simulink model "gm_HFMA_4B_1_5_9_13"  (R2026b)
settings: Solver=FixedStepDiscrete  StopTime=stopTime  FixedStep=1.953125e-06
PreLoadFcn:
  | load('a_luts.mat')
undefined symbols (not defined in the file or in its folder): Ts
libraries: simulink x202, simulink_need_slupdate x99, hdlsllib x91
(part 15 of 20)

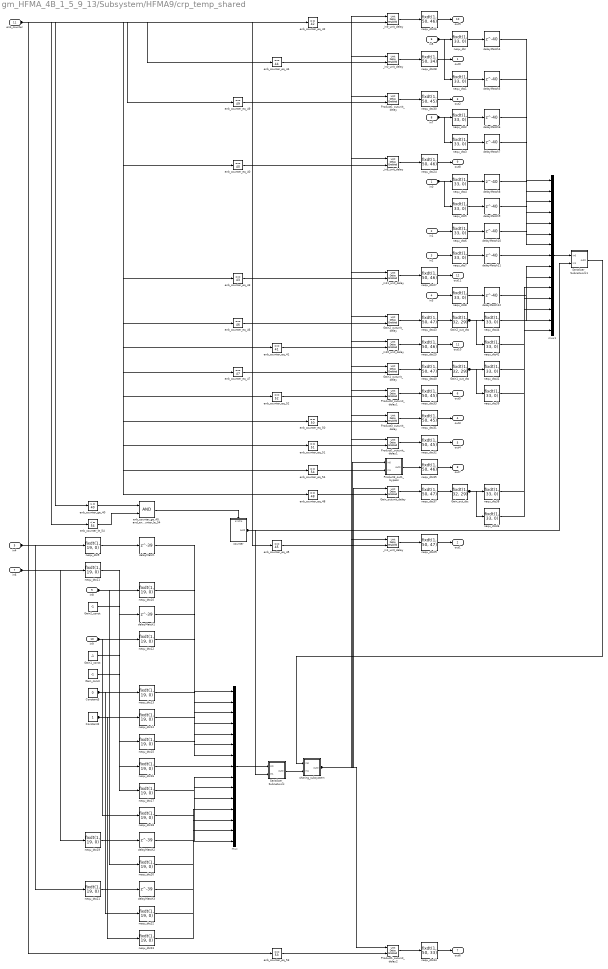
== system gm_HFMA_4B_1_5_9_13/Subsystem/HFMA9/crp_temp_shared ==
  in0 : Inport  OutDataTypeStr=fixdt(1,32,30,'DataTypeOverride', 'Off')  PortDimensions=1  SampleTime=1.953125e-06
  in1 : Inport  Port=2  OutDataTypeStr=fixdt(1,32,30,'DataTypeOverride', 'Off')  PortDimensions=1  SampleTime=1.953125e-06
  in2 : Inport  Port=3  OutDataTypeStr=fixdt(1,32,30,'DataTypeOverride', 'Off')  PortDimensions=1  SampleTime=1.953125e-06
  in3 : Inport  Port=4  OutDataTypeStr=fixdt(1,32,30,'DataTypeOverride', 'Off')  PortDimensions=1  SampleTime=1.953125e-06
  in4 : Inport  Port=5  OutDataTypeStr=fixdt(1,18,16,'DataTypeOverride', 'Off')  PortDimensions=1  SampleTime=1.953125e-06
  in5 : Inport  Port=6  OutDataTypeStr=fixdt(1,32,30,'DataTypeOverride', 'Off')  PortDimensions=1  SampleTime=1.953125e-06
  in6 : Inport  Port=7  OutDataTypeStr=fixdt(1,18,16,'DataTypeOverride', 'Off')  PortDimensions=1  SampleTime=1.953125e-06
  in7 : Inport  Port=8  OutDataTypeStr=fixdt(1,32,30,'DataTypeOverride', 'Off')  PortDimensions=1  SampleTime=1.953125e-06
  in8 : Inport  Port=9  OutDataTypeStr=fixdt(1,18,16,'DataTypeOverride', 'Off')  PortDimensions=1  SampleTime=1.953125e-06
  in9 : Inport  Port=10  OutDataTypeStr=fixdt(1,18,16,'DataTypeOverride', 'Off')  PortDimensions=1  SampleTime=1.953125e-06
  enb_counter : Inport  Port=11  OutDataTypeStr=fixdt(0,6,0,'DataTypeOverride', 'Off')  PortDimensions=1  SampleTime=1.953125e-06
  Constant2 : Constant  OutDataTypeStr=fixdt(0, 18, 17)  SampleTime=1.953125e-06
  Constant3 : Constant  Value=0  OutDataTypeStr=fixdt(1, 18, 4)  SampleTime=1.953125e-06
  Gain1_const : Constant  Value=-1  OutDataTypeStr=fixdt(1, 18, 17)  SampleTime=1.953125e-06
  Gain1_out_dtc : DataTypeConversion  OutDataTypeStr=fixdt(1, 32, 29)  SampleTime=1.953125e-06  RndMeth=Floor
  Gain1_outunit_delay : simulink_need_slupdate/Unit Delay Enabled  vinit=0.0  tsamp=-1
  Gain2_const : Constant  Value=-1  OutDataTypeStr=fixdt(1, 18, 17)  SampleTime=1.953125e-06
  Gain2_out_dtc : DataTypeConversion  OutDataTypeStr=fixdt(1, 32, 29)  SampleTime=1.953125e-06  RndMeth=Floor
  Gain2_outunit_delay : simulink_need_slupdate/Unit Delay Enabled  vinit=0.0  tsamp=-1
  Gain_const : Constant  Value=-1  OutDataTypeStr=fixdt(1, 18, 17)  SampleTime=1.953125e-06
  Gain_out_dtc : DataTypeConversion  OutDataTypeStr=fixdt(1, 32, 29)  SampleTime=1.953125e-06  RndMeth=Floor
  Gain_outunit_delay : simulink_need_slupdate/Unit Delay Enabled  vinit=0.0  tsamp=-1
  Product1_outunit_delay : simulink_need_slupdate/Unit Delay Enabled  vinit=0.0  tsamp=-1
  Product1_outunit_delay1 : simulink_need_slupdate/Unit Delay Enabled  vinit=0.0  tsamp=-1
  Product1_outunit_delay2 : simulink_need_slupdate/Unit Delay Enabled  vinit=0.0  tsamp=-1
  Product3_out1_bypass : Subsystem
  Product3_outunit_delay : simulink_need_slupdate/Unit Delay Enabled  vinit=0.0  tsamp=-1
  Product3_outunit_delay1 : simulink_need_slupdate/Unit Delay Enabled  vinit=0.0  tsamp=-1
  Serializer_Subnetwork : Subsystem
  Serializer_Subnetwork1 : Subsystem
  _in0_unit_delay : simulink_need_slupdate/Unit Delay Enabled  vinit=0.0  tsamp=-1
  _in10_unit_delay : simulink_need_slupdate/Unit Delay Enabled  vinit=0.0  tsamp=-1
  _in11_unit_delay : simulink_need_slupdate/Unit Delay Enabled  vinit=0.0  tsamp=-1
  _in1_unit_delay : simulink_need_slupdate/Unit Delay Enabled  vinit=0.0  tsamp=-1
  _in8_unit_delay : simulink_need_slupdate/Unit Delay Enabled  vinit=0.0  tsamp=-1
  _in9_unit_delay : simulink_need_slupdate/Unit Delay Enabled  vinit=0.0  tsamp=-1
  counter : Subsystem
  delayMatch{,1..3} (4 alike) : Delay  DelayLength=39  InitialCondition=0  SampleTime=1.953125e-06
  delayMatch{4..12} (9 alike) : Delay  DelayLength=40  InitialCondition=0  SampleTime=1.953125e-06
  enb_counter_eq_40 : simulink/Logic and Bit Operations/Compare To Constant  relop===  const=40  OutDataTypeStr=boolean
  enb_counter_eq_41 : simulink/Logic and Bit Operations/Compare To Constant  relop===  const=41  OutDataTypeStr=boolean
  enb_counter_eq_42 : simulink/Logic and Bit Operations/Compare To Constant  relop===  const=42  OutDataTypeStr=boolean
  enb_counter_eq_43 : simulink/Logic and Bit Operations/Compare To Constant  relop===  const=43  OutDataTypeStr=boolean
  enb_counter_eq_44 : simulink/Logic and Bit Operations/Compare To Constant  relop===  const=44  OutDataTypeStr=boolean
  enb_counter_eq_45 : simulink/Logic and Bit Operations/Compare To Constant  relop===  const=45  OutDataTypeStr=boolean
  enb_counter_eq_46 : simulink/Logic and Bit Operations/Compare To Constant  relop===  const=46  OutDataTypeStr=boolean
  enb_counter_eq_47 : simulink/Logic and Bit Operations/Compare To Constant  relop===  const=47  OutDataTypeStr=boolean
  enb_counter_eq_48 : simulink/Logic and Bit Operations/Compare To Constant  relop===  const=48  OutDataTypeStr=boolean
  enb_counter_eq_49 : simulink/Logic and Bit Operations/Compare To Constant  relop===  const=49  OutDataTypeStr=boolean
  enb_counter_eq_50 : simulink/Logic and Bit Operations/Compare To Constant  relop===  const=50  OutDataTypeStr=boolean
  enb_counter_eq_51 : simulink/Logic and Bit Operations/Compare To Constant  relop===  const=51  OutDataTypeStr=boolean
  enb_counter_eq_52 : simulink/Logic and Bit Operations/Compare To Constant  relop===  const=52  OutDataTypeStr=boolean
  enb_counter_eq_53 : simulink/Logic and Bit Operations/Compare To Constant  relop===  const=53  OutDataTypeStr=boolean
  enb_counter_eq_54 : simulink/Logic and Bit Operations/Compare To Constant  relop===  const=54  OutDataTypeStr=boolean
  enb_counter_ge_40 : simulink/Logic and Bit Operations/Compare To Constant  relop=>=  const=40  OutDataTypeStr=boolean
  enb_counter_ge_40_and_enb_counter_le_54 : Logic  AllPortsSameDT=off  OutDataTypeStr=boolean  SampleTime=1.953125e-06
  enb_counter_le_54 : simulink/Logic and Bit Operations/Compare To Constant  relop=<=  const=54  OutDataTypeStr=boolean
  mux : Mux  Inputs=15
  mux1 : Mux  Inputs=15
  nequ_dtc{,1..8,36,38..39,41..42,44} (15 alike) : DataTypeConversion  OutDataTypeStr=fixdt(1, 33, 0)  ConvertRealWorld=Stored Integer (SI)  SampleTime=1.953125e-06  SaturateOnIntegerOverflow=off  RndMeth=Floor
  nequ_dtc{9..23} (15 alike) : DataTypeConversion  OutDataTypeStr=fixdt(1, 19, 0)  ConvertRealWorld=Stored Integer (SI)  SampleTime=1.953125e-06  SaturateOnIntegerOverflow=off  RndMeth=Floor
  nequ_dtc{24..27,35} (5 alike) : DataTypeConversion  OutDataTypeStr=fixdt(1, 50, 46)  ConvertRealWorld=Stored Integer (SI)  SampleTime=1.953125e-06  SaturateOnIntegerOverflow=off  RndMeth=Floor
  nequ_dtc28 : DataTypeConversion  OutDataTypeStr=fixdt(1, 50, 34)  ConvertRealWorld=Stored Integer (SI)  SampleTime=1.953125e-06  SaturateOnIntegerOverflow=off  RndMeth=Floor
  nequ_dtc{29,37,40,43} (4 alike) : DataTypeConversion  OutDataTypeStr=fixdt(1, 50, 47)  ConvertRealWorld=Stored Integer (SI)  SampleTime=1.953125e-06  SaturateOnIntegerOverflow=off  RndMeth=Floor
  nequ_dtc{30..33} (4 alike) : DataTypeConversion  OutDataTypeStr=fixdt(1, 50, 45)  ConvertRealWorld=Stored Integer (SI)  SampleTime=1.953125e-06  SaturateOnIntegerOverflow=off  RndMeth=Floor
  nequ_dtc34 : DataTypeConversion  OutDataTypeStr=fixdt(1, 50, 33)  ConvertRealWorld=Stored Integer (SI)  SampleTime=1.953125e-06  SaturateOnIntegerOverflow=off  RndMeth=Floor
  sharing_subsystem : Subsystem
  out0 : Outport  OutDataTypeStr=fixdt(1,50,34,'DataTypeOverride', 'Off')  PortDimensions=1  SampleTime=1.953125e-06
  out1 : Outport  Port=2  OutDataTypeStr=fixdt(1,50,47,'DataTypeOverride', 'Off')  PortDimensions=1  SampleTime=1.953125e-06
  out2 : Outport  Port=3  OutDataTypeStr=fixdt(1,50,45,'DataTypeOverride', 'Off')  PortDimensions=1  SampleTime=1.953125e-06
  out3 : Outport  Port=4  OutDataTypeStr=fixdt(1,50,45,'DataTypeOverride', 'Off')  PortDimensions=1  SampleTime=1.953125e-06
  out4 : Outport  Port=5  OutDataTypeStr=fixdt(1,50,45,'DataTypeOverride', 'Off')  PortDimensions=1  SampleTime=1.953125e-06
  out5 : Outport  Port=6  OutDataTypeStr=fixdt(1,50,45,'DataTypeOverride', 'Off')  PortDimensions=1  SampleTime=1.953125e-06
  out6 : Outport  Port=7  OutDataTypeStr=fixdt(1,50,33,'DataTypeOverride', 'Off')  PortDimensions=1  SampleTime=1.953125e-06
  out7 : Outport  Port=8  OutDataTypeStr=fixdt(1,50,46,'DataTypeOverride', 'Off')  PortDimensions=1  SampleTime=1.953125e-06
  out8 : Outport  Port=9  OutDataTypeStr=fixdt(1,50,46,'DataTypeOverride', 'Off')  PortDimensions=1  SampleTime=1.953125e-06
  out9 : Outport  Port=10  OutDataTypeStr=fixdt(1,50,46,'DataTypeOverride', 'Off')  PortDimensions=1  SampleTime=1.953125e-06
  out10 : Outport  Port=11  OutDataTypeStr=fixdt(1,50,46,'DataTypeOverride', 'Off')  PortDimensions=1  SampleTime=1.953125e-06
  out11 : Outport  Port=12  OutDataTypeStr=fixdt(1,50,46,'DataTypeOverride', 'Off')  PortDimensions=1  SampleTime=1.953125e-06
  wires:
  nequ_dtc30/1 -> out2/1
  Product3_outunit_delay1/1 -> nequ_dtc33/1
  enb_counter_eq_48/1 -> Gain_outunit_delay/2
  nequ_dtc9/1 -> delayMatch/1
  Product3_out1_bypass/1(out0) -> nequ_dtc35/1
  Gain_outunit_delay/1 -> nequ_dtc37/1
  nequ_dtc11/1 -> delayMatch1/1
  Gain2_outunit_delay/1 -> nequ_dtc43/1
  nequ_dtc13/1 -> mux/5
  enb_counter_le_54/1 -> enb_counter_ge_40_and_enb_counter_le_54/2
  enb_counter_eq_50/1 -> Product3_outunit_delay/2
  nequ_dtc19/1 -> delayMatch2/1
  nequ_dtc21/1 -> delayMatch3/1
  enb_counter_ge_40/1 -> enb_counter_ge_40_and_enb_counter_le_54/1
  in3/1 -> nequ_dtc8/1
  nequ_dtc38/1 -> mux1/14
  nequ_dtc43/1 -> Gain2_out_dtc/1
  enb_counter_eq_42/1 -> _in9_unit_delay/2
  Serializer_Subnetwork/1(out0) -> sharing_subsystem/2(in1)
  delayMatch5/1 -> mux1/2
  enb_counter_eq_54/1 -> Product3_out1_bypass/2(in1)
  Gain_out_dtc/1 -> nequ_dtc36/1, nequ_dtc38/1
  in1/1 -> nequ_dtc6/1
  enb_counter_eq_51/1 -> Product1_outunit_delay1/2
  nequ_dtc44/1 -> mux1/10
  enb_counter_eq_46/1 -> Gain2_outunit_delay/2
  nequ_dtc4/1 -> delayMatch8/1
  in6/1 -> nequ_dtc11/1, nequ_dtc19/1
  nequ_dtc39/1 -> mux1/13
  nequ_dtc40/1 -> Gain1_out_dtc/1
  nequ_dtc27/1 -> out11/1
  nequ_dtc29/1 -> out1/1
  enb_counter/1 -> enb_counter_eq_53/1, enb_counter_eq_52/1, enb_counter_eq_50/1, enb_counter_eq_49/1, enb_counter_eq_48/1, enb_counter_eq_47/1, enb_counter_eq_46/1, enb_counter_eq_45/1, enb_counter_eq_41/1, enb_counter_eq_54/1, enb_counter_eq_44/1, enb_counter_eq_42/1, enb_counter_eq_40/1, enb_counter_eq_51/1, enb_counter_le_54/1, enb_counter_ge_40/1, enb_counter_eq_43/1
  nequ_dtc42/1 -> mux1/11
  nequ_dtc41/1 -> mux1/12
  delayMatch7/1 -> mux1/4
  delayMatch9/1 -> mux1/6
  Product1_outunit_delay2/1 -> nequ_dtc34/1
  Gain1_outunit_delay/1 -> nequ_dtc40/1
  nequ_dtc37/1 -> Gain_out_dtc/1
  Product3_outunit_delay/1 -> nequ_dtc31/1
  Product1_outunit_delay/1 -> nequ_dtc30/1
  nequ_dtc6/1 -> delayMatch10/1
  nequ_dtc8/1 -> delayMatch12/1
  mux1/1 -> Serializer_Subnetwork1/1(in0)
  nequ_dtc36/1 -> mux1/15
  nequ_dtc3/1 -> delayMatch7/1
  nequ_dtc5/1 -> delayMatch9/1
  delayMatch4/1 -> mux1/1
  delayMatch6/1 -> mux1/3
  delayMatch12/1 -> mux1/9
  delayMatch11/1 -> mux1/8
  Serializer_Subnetwork1/1(out0) -> sharing_subsystem/1(in0)
  delayMatch10/1 -> mux1/7
  _in1_unit_delay/1 -> nequ_dtc29/1
  delayMatch8/1 -> mux1/5
  Gain1_out_dtc/1 -> nequ_dtc41/1, nequ_dtc39/1
  nequ_dtc7/1 -> delayMatch11/1
  Gain1_const/1 -> nequ_dtc16/1
  nequ_dtc/1 -> delayMatch4/1
  sharing_subsystem/1(out0) -> Gain2_outunit_delay/1, Gain1_outunit_delay/1, Gain_outunit_delay/1, _in1_unit_delay/1, _in0_unit_delay/1, _in11_unit_delay/1, _in9_unit_delay/1, _in10_unit_delay/1, _in8_unit_delay/1, Product1_outunit_delay2/1, Product3_outunit_delay1/1, Product1_outunit_delay1/1, Product1_outunit_delay/1, Product3_out1_bypass/1(in0), Product3_outunit_delay/1
  nequ_dtc2/1 -> delayMatch6/1
  _in0_unit_delay/1 -> nequ_dtc28/1
  nequ_dtc1/1 -> delayMatch5/1
  nequ_dtc23/1 -> mux/15
  Product1_outunit_delay1/1 -> nequ_dtc32/1
  nequ_dtc28/1 -> out0/1
  _in11_unit_delay/1 -> nequ_dtc27/1
  nequ_dtc34/1 -> out6/1
  _in9_unit_delay/1 -> nequ_dtc26/1
  nequ_dtc26/1 -> out9/1
  _in10_unit_delay/1 -> nequ_dtc25/1
  nequ_dtc20/1 -> mux/12
  nequ_dtc25/1 -> out10/1
  mux/1 -> Serializer_Subnetwork/1(in0)
  _in8_unit_delay/1 -> nequ_dtc24/1
  nequ_dtc24/1 -> out8/1
  in5/1 -> nequ_dtc1/1, nequ_dtc/1
  nequ_dtc22/1 -> mux/14
  delayMatch3/1 -> mux/13
  delayMatch2/1 -> mux/11
  nequ_dtc18/1 -> mux/10
  nequ_dtc17/1 -> mux/9
  nequ_dtc16/1 -> mux/8
  nequ_dtc15/1 -> mux/7
  nequ_dtc14/1 -> mux/6
  nequ_dtc12/1 -> mux/4
  delayMatch1/1 -> mux/3
  nequ_dtc10/1 -> mux/2
  delayMatch/1 -> mux/1
  in2/1 -> nequ_dtc7/1
  nequ_dtc35/1 -> out7/1
  nequ_dtc33/1 -> out5/1
  nequ_dtc32/1 -> out4/1
  nequ_dtc31/1 -> out3/1
  Gain_const/1 -> nequ_dtc17/1
  Gain2_const/1 -> nequ_dtc15/1
  enb_counter_ge_40_and_enb_counter_le_54/1 -> counter/Enable
  Constant2/1 -> nequ_dtc14/1, nequ_dtc23/1
  counter/1(out0) -> Serializer_Subnetwork1/2(in1), Serializer_Subnetwork/2(in1)
  in9/1 -> nequ_dtc18/1, nequ_dtc12/1
  Gain2_out_dtc/1 -> nequ_dtc42/1, nequ_dtc44/1
  Constant3/1 -> nequ_dtc13/1, nequ_dtc22/1
  in0/1 -> nequ_dtc5/1, nequ_dtc4/1
  in8/1 -> nequ_dtc20/1, nequ_dtc10/1
  in7/1 -> nequ_dtc3/1, nequ_dtc2/1
  in4/1 -> nequ_dtc21/1, nequ_dtc9/1
  enb_counter_eq_53/1 -> Product1_outunit_delay2/2
  enb_counter_eq_49/1 -> Product1_outunit_delay/2
  enb_counter_eq_40/1 -> _in8_unit_delay/2
  enb_counter_eq_43/1 -> _in11_unit_delay/2
  enb_counter_eq_47/1 -> Gain1_outunit_delay/2
  enb_counter_eq_41/1 -> _in10_unit_delay/2
  enb_counter_eq_52/1 -> Product3_outunit_delay1/2
  enb_counter_eq_44/1 -> _in0_unit_delay/2
  enb_counter_eq_45/1 -> _in1_unit_delay/2

== system gm_HFMA_4B_1_5_9_13/Subsystem/HFMA9/crp_temp_shared1 ==
  in0 : Inport  OutDataTypeStr=fixdt(1,20,17,'DataTypeOverride', 'Off')  PortDimensions=1  SampleTime=1.953125e-06
  in1 : Inport  Port=2  OutDataTypeStr=fixdt(1,18,16,'DataTypeOverride', 'Off')  PortDimensions=1  SampleTime=1.953125e-06
  in2 : Inport  Port=3  OutDataTypeStr=fixdt(1,18,16,'DataTypeOverride', 'Off')  PortDimensions=1  SampleTime=1.953125e-06
  in3 : Inport  Port=4  OutDataTypeStr=fixdt(1,20,17,'DataTypeOverride', 'Off')  PortDimensions=1  SampleTime=1.953125e-06
  in4 : Inport  Port=5  OutDataTypeStr=fixdt(1,18,16,'DataTypeOverride', 'Off')  PortDimensions=1  SampleTime=1.953125e-06
  in5 : Inport  Port=6  OutDataTypeStr=fixdt(1,20,17,'DataTypeOverride', 'Off')  PortDimensions=1  SampleTime=1.953125e-06
  in6 : Inport  Port=7  OutDataTypeStr=fixdt(1,18,16,'DataTypeOverride', 'Off')  PortDimensions=1  SampleTime=1.953125e-06
  in7 : Inport  Port=8  OutDataTypeStr=fixdt(1,18,16,'DataTypeOverride', 'Off')  PortDimensions=1  SampleTime=1.953125e-06
  in8 : Inport  Port=9  OutDataTypeStr=fixdt(1,20,17,'DataTypeOverride', 'Off')  PortDimensions=1  SampleTime=1.953125e-06
  in9 : Inport  Port=10  OutDataTypeStr=fixdt(1,18,16,'DataTypeOverride', 'Off')  PortDimensions=1  SampleTime=1.953125e-06
  in10 : Inport  Port=11  OutDataTypeStr=fixdt(1,18,16,'DataTypeOverride', 'Off')  PortDimensions=1  SampleTime=1.953125e-06
  in11 : Inport  Port=12  OutDataTypeStr=fixdt(1,18,16,'DataTypeOverride', 'Off')  PortDimensions=1  SampleTime=1.953125e-06
  enb_counter : Inport  Port=13  OutDataTypeStr=fixdt(0,6,0,'DataTypeOverride', 'Off')  PortDimensions=1  SampleTime=1.953125e-06
  Product1 : Product  Inputs=**  OutDataTypeStr=fixdt(1, 38, 33)  SampleTime=1.953125e-06
  Serializer_Subnetwork : Subsystem
  Serializer_Subnetwork1 : Subsystem
  counter : Subsystem
  counter_matching_delay : Delay  DelayLength=15  InitialCondition=0  SampleTime=1.953125e-06
  delayMatch : Delay  DelayLength=15  InitialCondition=0  SampleTime=1.953125e-06
  demux : Demux  Outputs=8
  enb_counter_eq_23 : simulink/Logic and Bit Operations/Compare To Constant  relop===  const=23  OutDataTypeStr=boolean
  enb_counter_ge_1 : simulink/Logic and Bit Operations/Compare To Constant  relop=>=  const=1  OutDataTypeStr=boolean
  enb_counter_ge_16 : simulink/Logic and Bit Operations/Compare To Constant  relop=>=  const=16  OutDataTypeStr=boolean
  enb_counter_ge_16_and_enb_counter_le_23 : Logic  AllPortsSameDT=off  OutDataTypeStr=boolean  SampleTime=1.953125e-06
  enb_counter_ge_1_and_enb_counter_le_8 : Logic  AllPortsSameDT=off  OutDataTypeStr=boolean  SampleTime=1.953125e-06
  enb_counter_le_23 : simulink/Logic and Bit Operations/Compare To Constant  relop=<=  const=23  OutDataTypeStr=boolean
  enb_counter_le_8 : simulink/Logic and Bit Operations/Compare To Constant  relop=<=  const=8  OutDataTypeStr=boolean
  mux : Mux  Inputs=8
  mux1 : Mux  Inputs=8
  tapped_delay : hdlsllib/Discrete/Tapped Delay Enabled Synchronous  vinit=0  samptime=-1  NumDelays=7  DelayOrder=Oldest  includeCurrent=on
  tapped_delay_outunit_delay : simulink_need_slupdate/Unit Delay Enabled  vinit=0.0  tsamp=-1
  out0 : Outport  OutDataTypeStr=fixdt(1,38,33,'DataTypeOverride', 'Off')  PortDimensions=1  SampleTime=1.953125e-06
  out1 : Outport  Port=2  OutDataTypeStr=fixdt(1,38,33,'DataTypeOverride', 'Off')  PortDimensions=1  SampleTime=1.953125e-06
  out2 : Outport  Port=3  OutDataTypeStr=fixdt(1,38,33,'DataTypeOverride', 'Off')  PortDimensions=1  SampleTime=1.953125e-06
  out3 : Outport  Port=4  OutDataTypeStr=fixdt(1,38,33,'DataTypeOverride', 'Off')  PortDimensions=1  SampleTime=1.953125e-06
  out4 : Outport  Port=5  OutDataTypeStr=fixdt(1,38,33,'DataTypeOverride', 'Off')  PortDimensions=1  SampleTime=1.953125e-06
  out5 : Outport  Port=6  OutDataTypeStr=fixdt(1,38,33,'DataTypeOverride', 'Off')  PortDimensions=1  SampleTime=1.953125e-06
  out6 : Outport  Port=7  OutDataTypeStr=fixdt(1,38,33,'DataTypeOverride', 'Off')  PortDimensions=1  SampleTime=1.953125e-06
  out7 : Outport  Port=8  OutDataTypeStr=fixdt(1,38,33,'DataTypeOverride', 'Off')  PortDimensions=1  SampleTime=1.953125e-06
  wires:
  in10/1 -> mux1/7
  enb_counter/1 -> enb_counter_le_23/1, enb_counter_eq_23/1, enb_counter_le_8/1, enb_counter_ge_1/1, enb_counter_ge_16/1
  in5/1 -> mux/8, mux/4
  in7/1 -> mux1/5
  enb_counter_ge_1/1 -> enb_counter_ge_1_and_enb_counter_le_8/1
  enb_counter_ge_1_and_enb_counter_le_8/1 -> counter/Enable
  enb_counter_le_8/1 -> enb_counter_ge_1_and_enb_counter_le_8/2
  enb_counter_ge_16/1 -> enb_counter_ge_16_and_enb_counter_le_23/1
  enb_counter_le_23/1 -> enb_counter_ge_16_and_enb_counter_le_23/2
  in2/1 -> mux1/2
  in1/1 -> mux1/1
  in4/1 -> mux1/3
  in6/1 -> mux1/4
  in9/1 -> mux1/6
  in11/1 -> mux1/8
  enb_counter_ge_16_and_enb_counter_le_23/1 -> tapped_delay/2
  in0/1 -> mux/2, mux/1
  in3/1 -> mux/3, mux/5
  in8/1 -> mux/7, mux/6
  counter/1(out0) -> Serializer_Subnetwork1/2(in1), counter_matching_delay/1
  mux1/1 -> Serializer_Subnetwork1/1(in0)
  mux/1 -> Serializer_Subnetwork/1(in0)
  counter_matching_delay/1 -> Serializer_Subnetwork/2(in1)
  Serializer_Subnetwork1/1(out0) -> delayMatch/1
  Serializer_Subnetwork/1(out0) -> Product1/1
  demux/7 -> out6/1
  delayMatch/1 -> Product1/2
  Product1/1 -> tapped_delay/1
  enb_counter_eq_23/1 -> tapped_delay_outunit_delay/2
  tapped_delay/1 -> tapped_delay_outunit_delay/1
  tapped_delay_outunit_delay/1 -> demux/1
  demux/3 -> out2/1
  demux/1 -> out0/1
  demux/2 -> out1/1
  demux/6 -> out5/1
  demux/4 -> out3/1
  demux/5 -> out4/1
  demux/8 -> out7/1

== system gm_HFMA_4B_1_5_9_13/Subsystem/HFMA9/crp_temp_shared2 ==
  in0 : Inport  OutDataTypeStr=fixdt(1,18,15,'DataTypeOverride', 'Off')  PortDimensions=1  SampleTime=1.953125e-06
  in1 : Inport  Port=2  OutDataTypeStr=fixdt(1,18,15,'DataTypeOverride', 'Off')  PortDimensions=1  SampleTime=1.953125e-06
  in2 : Inport  Port=3  OutDataTypeStr=fixdt(1,18,15,'DataTypeOverride', 'Off')  PortDimensions=1  SampleTime=1.953125e-06
  in3 : Inport  Port=4  OutDataTypeStr=fixdt(1,18,15,'DataTypeOverride', 'Off')  PortDimensions=1  SampleTime=1.953125e-06
  in4 : Inport  Port=5  OutDataTypeStr=fixdt(1,18,16,'DataTypeOverride', 'Off')  PortDimensions=1  SampleTime=1.953125e-06
  in5 : Inport  Port=6  OutDataTypeStr=fixdt(1,18,16,'DataTypeOverride', 'Off')  PortDimensions=1  SampleTime=1.953125e-06
  in6 : Inport  Port=7  OutDataTypeStr=fixdt(1,18,14,'DataTypeOverride', 'Off')  PortDimensions=1  SampleTime=1.953125e-06
  in7 : Inport  Port=8  OutDataTypeStr=fixdt(1,18,14,'DataTypeOverride', 'Off')  PortDimensions=1  SampleTime=1.953125e-06
  in8 : Inport  Port=9  OutDataTypeStr=fixdt(1,18,14,'DataTypeOverride', 'Off')  PortDimensions=1  SampleTime=1.953125e-06
  in9 : Inport  Port=10  OutDataTypeStr=fixdt(1,18,14,'DataTypeOverride', 'Off')  PortDimensions=1  SampleTime=1.953125e-06
  enb_counter : Inport  Port=11  OutDataTypeStr=fixdt(0,6,0,'DataTypeOverride', 'Off')  PortDimensions=1  SampleTime=1.953125e-06
  Gain : Product  Inputs=**  OutDataTypeStr=fixdt(1, 36, 0)  SampleTime=1.953125e-06
  Gain1_const : Constant  Value=-1  OutDataTypeStr=fixdt(1, 18, 17)  SampleTime=1.953125e-06
  Gain_const{,1..3} (4 alike) : Constant  Value=-2  OutDataTypeStr=fixdt(1, 18, 16)  SampleTime=1.953125e-06
  Gain_const4 : Constant  Value=-1  OutDataTypeStr=fixdt(1, 18, 17)  SampleTime=1.953125e-06
  Serializer_Subnetwork : Subsystem
  Serializer_Subnetwork1 : Subsystem
  b0_1_const : Constant  Value=0.001172125339508056640625  OutDataTypeStr=fixdt(1, 18, 26)  SampleTime=1.953125e-06
  b0_1_const1 : Constant  Value=0.001172125339508056640625  OutDataTypeStr=fixdt(1, 18, 26)  SampleTime=1.953125e-06
  b0_1_const2 : Constant  Value=0.001172125339508056640625  OutDataTypeStr=fixdt(1, 18, 26)  SampleTime=1.953125e-06
  b1_1_const : Constant  Value=0.00234425067901611328125  OutDataTypeStr=fixdt(1, 18, 25)  SampleTime=1.953125e-06
  b1_1_const1 : Constant  Value=0.00234425067901611328125  OutDataTypeStr=fixdt(1, 18, 25)  SampleTime=1.953125e-06
  b1_1_const2 : Constant  Value=0.00234425067901611328125  OutDataTypeStr=fixdt(1, 18, 25)  SampleTime=1.953125e-06
  b2_1_const{,1..3} (4 alike) : Constant  Value=0.001172125339508056640625  OutDataTypeStr=fixdt(1, 18, 26)  SampleTime=1.953125e-06
  counter : Subsystem
  counter_matching_delay : Delay  DelayLength=24  InitialCondition=0  SampleTime=1.953125e-06
  delayMatch : Delay  DelayLength=23  InitialCondition=0  SampleTime=1.953125e-06
  delayMatch1 : Delay  DelayLength=23  InitialCondition=0  SampleTime=1.953125e-06
  delayMatch2 : Delay  DelayLength=24  InitialCondition=0  SampleTime=1.953125e-06
  demux : Demux  Outputs=16
  enb_counter_eq_39 : simulink/Logic and Bit Operations/Compare To Constant  relop===  const=39  OutDataTypeStr=boolean
  enb_counter_ge_24 : simulink/Logic and Bit Operations/Compare To Constant  relop=>=  const=24  OutDataTypeStr=boolean
  enb_counter_ge_24_and_enb_counter_le_39 : Logic  AllPortsSameDT=off  OutDataTypeStr=boolean  SampleTime=1.953125e-06
  enb_counter_le_15 : simulink/Logic and Bit Operations/Compare To Constant  relop=<=  const=15  OutDataTypeStr=boolean
  enb_counter_le_39 : simulink/Logic and Bit Operations/Compare To Constant  relop=<=  const=39  OutDataTypeStr=boolean
  mux : Mux  Inputs=16
  mux1 : Mux  Inputs=16
  nequ_dtc{,1..31} (32 alike) : DataTypeConversion  OutDataTypeStr=fixdt(1, 18, 0)  ConvertRealWorld=Stored Integer (SI)  SampleTime=1.953125e-06  SaturateOnIntegerOverflow=off  RndMeth=Floor
  nequ_dtc{32..35} (4 alike) : DataTypeConversion  OutDataTypeStr=fixdt(1, 36, 31)  ConvertRealWorld=Stored Integer (SI)  SampleTime=1.953125e-06  SaturateOnIntegerOverflow=off  RndMeth=Floor
  nequ_dtc36 : DataTypeConversion  OutDataTypeStr=fixdt(1, 36, 33)  ConvertRealWorld=Stored Integer (SI)  SampleTime=1.953125e-06  SaturateOnIntegerOverflow=off  RndMeth=Floor
  nequ_dtc37 : DataTypeConversion  OutDataTypeStr=fixdt(1, 36, 33)  ConvertRealWorld=Stored Integer (SI)  SampleTime=1.953125e-06  SaturateOnIntegerOverflow=off  RndMeth=Floor
  nequ_dtc{38..39,41..42,44..45,47} (7 alike) : DataTypeConversion  OutDataTypeStr=fixdt(1, 36, 40)  ConvertRealWorld=Stored Integer (SI)  SampleTime=1.953125e-06  SaturateOnIntegerOverflow=off  RndMeth=Floor
  nequ_dtc40 : DataTypeConversion  OutDataTypeStr=fixdt(1, 36, 39)  ConvertRealWorld=Stored Integer (SI)  SampleTime=1.953125e-06  SaturateOnIntegerOverflow=off  RndMeth=Floor
  nequ_dtc43 : DataTypeConversion  OutDataTypeStr=fixdt(1, 36, 39)  ConvertRealWorld=Stored Integer (SI)  SampleTime=1.953125e-06  SaturateOnIntegerOverflow=off  RndMeth=Floor
  nequ_dtc46 : DataTypeConversion  OutDataTypeStr=fixdt(1, 36, 39)  ConvertRealWorld=Stored Integer (SI)  SampleTime=1.953125e-06  SaturateOnIntegerOverflow=off  RndMeth=Floor
  tapped_delay : hdlsllib/Discrete/Tapped Delay Enabled Synchronous  vinit=0  samptime=-1  NumDelays=15  DelayOrder=Oldest  includeCurrent=on
  tapped_delay_outunit_delay : simulink_need_slupdate/Unit Delay Enabled  vinit=0.0  tsamp=-1
  out0 : Outport  OutDataTypeStr=fixdt(1,36,31,'DataTypeOverride', 'Off')  PortDimensions=1  SampleTime=1.953125e-06
  out1 : Outport  Port=2  OutDataTypeStr=fixdt(1,36,31,'DataTypeOverride', 'Off')  PortDimensions=1  SampleTime=1.953125e-06
  out2 : Outport  Port=3  OutDataTypeStr=fixdt(1,36,31,'DataTypeOverride', 'Off')  PortDimensions=1  SampleTime=1.953125e-06
  out3 : Outport  Port=4  OutDataTypeStr=fixdt(1,36,31,'DataTypeOverride', 'Off')  PortDimensions=1  SampleTime=1.953125e-06
  out4 : Outport  Port=5  OutDataTypeStr=fixdt(1,36,33,'DataTypeOverride', 'Off')  PortDimensions=1  SampleTime=1.953125e-06
  out5 : Outport  Port=6  OutDataTypeStr=fixdt(1,36,33,'DataTypeOverride', 'Off')  PortDimensions=1  SampleTime=1.953125e-06
  out6 : Outport  Port=7  OutDataTypeStr=fixdt(1,36,40,'DataTypeOverride', 'Off')  PortDimensions=1  SampleTime=1.953125e-06
  out7 : Outport  Port=8  OutDataTypeStr=fixdt(1,36,40,'DataTypeOverride', 'Off')  PortDimensions=1  SampleTime=1.953125e-06
  out8 : Outport  Port=9  OutDataTypeStr=fixdt(1,36,39,'DataTypeOverride', 'Off')  PortDimensions=1  SampleTime=1.953125e-06
  out9 : Outport  Port=10  OutDataTypeStr=fixdt(1,36,40,'DataTypeOverride', 'Off')  PortDimensions=1  SampleTime=1.953125e-06
  out10 : Outport  Port=11  OutDataTypeStr=fixdt(1,36,40,'DataTypeOverride', 'Off')  PortDimensions=1  SampleTime=1.953125e-06
  out11 : Outport  Port=12  OutDataTypeStr=fixdt(1,36,39,'DataTypeOverride', 'Off')  PortDimensions=1  SampleTime=1.953125e-06
  out12 : Outport  Port=13  OutDataTypeStr=fixdt(1,36,40,'DataTypeOverride', 'Off')  PortDimensions=1  SampleTime=1.953125e-06
  out13 : Outport  Port=14  OutDataTypeStr=fixdt(1,36,40,'DataTypeOverride', 'Off')  PortDimensions=1  SampleTime=1.953125e-06
  out14 : Outport  Port=15  OutDataTypeStr=fixdt(1,36,39,'DataTypeOverride', 'Off')  PortDimensions=1  SampleTime=1.953125e-06
  out15 : Outport  Port=16  OutDataTypeStr=fixdt(1,36,40,'DataTypeOverride', 'Off')  PortDimensions=1  SampleTime=1.953125e-06
  wires:
  Gain_const/1 -> nequ_dtc/1
  Gain_const1/1 -> nequ_dtc1/1
  Gain_const2/1 -> nequ_dtc2/1
  Gain_const3/1 -> nequ_dtc3/1
  Gain1_const/1 -> nequ_dtc4/1
  Gain_const4/1 -> nequ_dtc5/1
  b2_1_const/1 -> nequ_dtc6/1
  b0_1_const/1 -> nequ_dtc7/1
  b1_1_const1/1 -> nequ_dtc11/1
  b0_1_const1/1 -> nequ_dtc10/1
  b2_1_const1/1 -> nequ_dtc9/1
  b1_1_const/1 -> nequ_dtc8/1
  b2_1_const3/1 -> nequ_dtc15/1
  b1_1_const2/1 -> nequ_dtc14/1
  b0_1_const2/1 -> nequ_dtc13/1
  b2_1_const2/1 -> nequ_dtc12/1
  enb_counter_ge_24/1 -> enb_counter_ge_24_and_enb_counter_le_39/1
  demux/2 -> nequ_dtc33/1
  in4/1 -> nequ_dtc20/1
  nequ_dtc4/1 -> mux/5
  nequ_dtc2/1 -> mux/3
  in5/1 -> nequ_dtc21/1
  nequ_dtc34/1 -> out2/1
  enb_counter/1 -> enb_counter_eq_39/1, enb_counter_le_39/1, enb_counter_le_15/1, enb_counter_ge_24/1
  nequ_dtc/1 -> mux/1
  in8/1 -> nequ_dtc30/1, nequ_dtc29/1, nequ_dtc28/1
  nequ_dtc1/1 -> mux/2
  nequ_dtc3/1 -> mux/4
  nequ_dtc5/1 -> mux/6
  nequ_dtc6/1 -> mux/7
  nequ_dtc9/1 -> mux/10
  nequ_dtc7/1 -> mux/8
  nequ_dtc8/1 -> mux/9
  nequ_dtc12/1 -> mux/13
  nequ_dtc10/1 -> mux/11
  nequ_dtc11/1 -> mux/12
  nequ_dtc13/1 -> mux/14
  nequ_dtc14/1 -> mux/15
  nequ_dtc15/1 -> mux/16
  in0/1 -> nequ_dtc16/1
  in3/1 -> nequ_dtc19/1
  in1/1 -> nequ_dtc17/1
  nequ_dtc42/1 -> out10/1
  in2/1 -> nequ_dtc18/1
  nequ_dtc22/1 -> mux1/7
  nequ_dtc20/1 -> delayMatch/1
  nequ_dtc21/1 -> delayMatch1/1
  demux/8 -> nequ_dtc39/1
  in6/1 -> nequ_dtc24/1, nequ_dtc23/1, nequ_dtc22/1
  enb_counter_le_15/1 -> counter/Enable
  in7/1 -> nequ_dtc27/1, nequ_dtc25/1, nequ_dtc26/1
  nequ_dtc16/1 -> mux1/1
  in9/1 -> nequ_dtc31/1
  nequ_dtc27/1 -> mux1/12
  nequ_dtc25/1 -> mux1/10
  enb_counter_le_39/1 -> enb_counter_ge_24_and_enb_counter_le_39/2
  mux/1 -> Serializer_Subnetwork/1(in0)
  nequ_dtc19/1 -> mux1/4
  counter_matching_delay/1 -> Serializer_Subnetwork1/2(in1)
  nequ_dtc17/1 -> mux1/2
  nequ_dtc18/1 -> mux1/3
  delayMatch/1 -> mux1/5
  delayMatch1/1 -> mux1/6
  nequ_dtc23/1 -> mux1/8
  counter/1(out0) -> counter_matching_delay/1, Serializer_Subnetwork/2(in1)
  nequ_dtc24/1 -> mux1/9
  nequ_dtc26/1 -> mux1/11
  nequ_dtc28/1 -> mux1/13
  nequ_dtc29/1 -> mux1/14
  enb_counter_ge_24_and_enb_counter_le_39/1 -> tapped_delay/2
  nequ_dtc30/1 -> mux1/15
  nequ_dtc31/1 -> mux1/16
  nequ_dtc39/1 -> out7/1
  Serializer_Subnetwork/1(out0) -> delayMatch2/1
  mux1/1 -> Serializer_Subnetwork1/1(in0)
  delayMatch2/1 -> Gain/1
  Serializer_Subnetwork1/1(out0) -> Gain/2
  Gain/1 -> tapped_delay/1
  enb_counter_eq_39/1 -> tapped_delay_outunit_delay/2
  tapped_delay/1 -> tapped_delay_outunit_delay/1
  tapped_delay_outunit_delay/1 -> demux/1
  demux/1 -> nequ_dtc32/1
  demux/3 -> nequ_dtc34/1
  demux/4 -> nequ_dtc35/1
  demux/5 -> nequ_dtc36/1
  demux/6 -> nequ_dtc37/1
  demux/7 -> nequ_dtc38/1
  demux/9 -> nequ_dtc40/1
  demux/10 -> nequ_dtc41/1
  demux/11 -> nequ_dtc42/1
  demux/12 -> nequ_dtc43/1
  demux/13 -> nequ_dtc44/1
  demux/14 -> nequ_dtc45/1
  demux/15 -> nequ_dtc46/1
  demux/16 -> nequ_dtc47/1
  nequ_dtc32/1 -> out0/1
  nequ_dtc33/1 -> out1/1
  nequ_dtc35/1 -> out3/1
  nequ_dtc36/1 -> out4/1
  nequ_dtc37/1 -> out5/1
  nequ_dtc38/1 -> out6/1
  nequ_dtc40/1 -> out8/1
  nequ_dtc41/1 -> out9/1
  nequ_dtc43/1 -> out11/1
  nequ_dtc44/1 -> out12/1
  nequ_dtc45/1 -> out13/1
  nequ_dtc46/1 -> out14/1
  nequ_dtc47/1 -> out15/1

== system gm_HFMA_4B_1_5_9_13/Subsystem/HFMA9/crp_temp_shared3 ==
  in0 : Inport  OutDataTypeStr=fixdt(1,18,14,'DataTypeOverride', 'Off')  PortDimensions=1  SampleTime=1.953125e-06
  in1 : Inport  Port=2  OutDataTypeStr=fixdt(1,18,14,'DataTypeOverride', 'Off')  PortDimensions=1  SampleTime=1.953125e-06
  in2 : Inport  Port=3  OutDataTypeStr=fixdt(1,18,14,'DataTypeOverride', 'Off')  PortDimensions=1  SampleTime=1.953125e-06
  in3 : Inport  Port=4  OutDataTypeStr=fixdt(1,18,14,'DataTypeOverride', 'Off')  PortDimensions=1  SampleTime=1.953125e-06
  in4 : Inport  Port=5  OutDataTypeStr=fixdt(1,18,14,'DataTypeOverride', 'Off')  PortDimensions=1  SampleTime=1.953125e-06
  in5 : Inport  Port=6  OutDataTypeStr=fixdt(1,18,16,'DataTypeOverride', 'Off')  PortDimensions=1  SampleTime=1.953125e-06
  enb_counter : Inport  Port=7  OutDataTypeStr=fixdt(0,6,0,'DataTypeOverride', 'Off')  PortDimensions=1  SampleTime=1.953125e-06
  Serializer_Subnetwork : Subsystem
  Serializer_Subnetwork1 : Subsystem
  b0_1 : Product  Inputs=**  OutDataTypeStr=fixdt(1, 36, 0)  SampleTime=1.953125e-06
  b0_1_const{,1..4} (5 alike) : Constant  Value=0.001172125339508056640625  OutDataTypeStr=fixdt(1, 18, 26)  SampleTime=1.953125e-06
  b0_2_const : Constant  Value=0.00121574103832244873046875  OutDataTypeStr=fixdt(1, 18, 26)  SampleTime=1.953125e-06
  b1_1_const{,1..4} (5 alike) : Constant  Value=0.00234425067901611328125  OutDataTypeStr=fixdt(1, 18, 25)  SampleTime=1.953125e-06
  b2_1_const{,1..3} (4 alike) : Constant  Value=0.001172125339508056640625  OutDataTypeStr=fixdt(1, 18, 26)  SampleTime=1.953125e-06
  b2_2_const : Constant  Value=0.00121574103832244873046875  OutDataTypeStr=fixdt(1, 18, 26)  SampleTime=1.953125e-06
  counter : Subsystem
  counter_matching_delay : Delay  DelayLength=64  InitialCondition=0  SampleTime=1.953125e-06
  delayMatch : Delay  DelayLength=16  InitialCondition=0  SampleTime=1.953125e-06
  delayMatch1 : Delay  DelayLength=16  InitialCondition=0  SampleTime=1.953125e-06
  delayMatch{3..17} (15 alike) : Delay  DelayLength=24  InitialCondition=0  SampleTime=1.953125e-06
  delayMatch2 : Delay  DelayLength=40  InitialCondition=0  SampleTime=1.953125e-06
  demux : Demux  Outputs=16
  enb_counter_eq_15 : simulink/Logic and Bit Operations/Compare To Constant  relop===  const=15  OutDataTypeStr=boolean
  enb_counter_le_15 : simulink/Logic and Bit Operations/Compare To Constant  relop=<=  const=15  OutDataTypeStr=boolean
  mux : Mux  Inputs=16
  mux1 : Mux  Inputs=16
  nequ_dtc{,1..31} (32 alike) : DataTypeConversion  OutDataTypeStr=fixdt(1, 18, 0)  ConvertRealWorld=Stored Integer (SI)  SampleTime=1.953125e-06  SaturateOnIntegerOverflow=off  RndMeth=Floor
  nequ_dtc{32,34..35,37..38,40..41,43..44} (9 alike) : DataTypeConversion  OutDataTypeStr=fixdt(1, 36, 40)  ConvertRealWorld=Stored Integer (SI)  SampleTime=1.953125e-06  SaturateOnIntegerOverflow=off  RndMeth=Floor
  nequ_dtc{33,36,39,42,45} (5 alike) : DataTypeConversion  OutDataTypeStr=fixdt(1, 36, 39)  ConvertRealWorld=Stored Integer (SI)  SampleTime=1.953125e-06  SaturateOnIntegerOverflow=off  RndMeth=Floor
  nequ_dtc46 : DataTypeConversion  OutDataTypeStr=fixdt(1, 36, 42)  ConvertRealWorld=Stored Integer (SI)  SampleTime=1.953125e-06  SaturateOnIntegerOverflow=off  RndMeth=Floor
  nequ_dtc47 : DataTypeConversion  OutDataTypeStr=fixdt(1, 36, 42)  ConvertRealWorld=Stored Integer (SI)  SampleTime=1.953125e-06  SaturateOnIntegerOverflow=off  RndMeth=Floor
  tapped_delay : hdlsllib/Discrete/Tapped Delay Enabled Synchronous  vinit=0  samptime=-1  NumDelays=15  DelayOrder=Oldest  includeCurrent=on
  tapped_delay_outunit_delay : simulink_need_slupdate/Unit Delay Enabled  vinit=0.0  tsamp=-1
  out0 : Outport  OutDataTypeStr=fixdt(1,36,40,'DataTypeOverride', 'Off')  PortDimensions=1  SampleTime=1.953125e-06
  out1 : Outport  Port=2  OutDataTypeStr=fixdt(1,36,39,'DataTypeOverride', 'Off')  PortDimensions=1  SampleTime=1.953125e-06
  out2 : Outport  Port=3  OutDataTypeStr=fixdt(1,36,40,'DataTypeOverride', 'Off')  PortDimensions=1  SampleTime=1.953125e-06
  out3 : Outport  Port=4  OutDataTypeStr=fixdt(1,36,40,'DataTypeOverride', 'Off')  PortDimensions=1  SampleTime=1.953125e-06
  out4 : Outport  Port=5  OutDataTypeStr=fixdt(1,36,39,'DataTypeOverride', 'Off')  PortDimensions=1  SampleTime=1.953125e-06
  out5 : Outport  Port=6  OutDataTypeStr=fixdt(1,36,40,'DataTypeOverride', 'Off')  PortDimensions=1  SampleTime=1.953125e-06
  out6 : Outport  Port=7  OutDataTypeStr=fixdt(1,36,40,'DataTypeOverride', 'Off')  PortDimensions=1  SampleTime=1.953125e-06
  out7 : Outport  Port=8  OutDataTypeStr=fixdt(1,36,39,'DataTypeOverride', 'Off')  PortDimensions=1  SampleTime=1.953125e-06
  out8 : Outport  Port=9  OutDataTypeStr=fixdt(1,36,40,'DataTypeOverride', 'Off')  PortDimensions=1  SampleTime=1.953125e-06
  out9 : Outport  Port=10  OutDataTypeStr=fixdt(1,36,40,'DataTypeOverride', 'Off')  PortDimensions=1  SampleTime=1.953125e-06
  out10 : Outport  Port=11  OutDataTypeStr=fixdt(1,36,39,'DataTypeOverride', 'Off')  PortDimensions=1  SampleTime=1.953125e-06
  out11 : Outport  Port=12  OutDataTypeStr=fixdt(1,36,40,'DataTypeOverride', 'Off')  PortDimensions=1  SampleTime=1.953125e-06
  out12 : Outport  Port=13  OutDataTypeStr=fixdt(1,36,40,'DataTypeOverride', 'Off')  PortDimensions=1  SampleTime=1.953125e-06
  out13 : Outport  Port=14  OutDataTypeStr=fixdt(1,36,39,'DataTypeOverride', 'Off')  PortDimensions=1  SampleTime=1.953125e-06
  out14 : Outport  Port=15  OutDataTypeStr=fixdt(1,36,42,'DataTypeOverride', 'Off')  PortDimensions=1  SampleTime=1.953125e-06
  out15 : Outport  Port=16  OutDataTypeStr=fixdt(1,36,42,'DataTypeOverride', 'Off')  PortDimensions=1  SampleTime=1.953125e-06
  wires:
  b0_1_const/1 -> nequ_dtc/1
  nequ_dtc2/1 -> mux/3
  nequ_dtc/1 -> mux/1
  b1_1_const/1 -> nequ_dtc1/1
  b2_1_const/1 -> nequ_dtc2/1
  b0_1_const1/1 -> nequ_dtc3/1
  b1_1_const1/1 -> nequ_dtc4/1
  b2_1_const2/1 -> nequ_dtc8/1
  b2_1_const1/1 -> nequ_dtc5/1
  b0_1_const2/1 -> nequ_dtc6/1
  b1_1_const2/1 -> nequ_dtc7/1
  b0_1_const4/1 -> nequ_dtc12/1
  b2_1_const3/1 -> nequ_dtc11/1
  b1_1_const3/1 -> nequ_dtc10/1
  b0_1_const3/1 -> nequ_dtc9/1
  nequ_dtc14/1 -> mux/15
  b0_2_const/1 -> nequ_dtc15/1
  nequ_dtc12/1 -> mux/13
  b2_2_const/1 -> nequ_dtc14/1
  b1_1_const4/1 -> nequ_dtc13/1
  in0/1 -> nequ_dtc17/1, nequ_dtc16/1
  in4/1 -> nequ_dtc29/1, nequ_dtc28/1, nequ_dtc27/1
  nequ_dtc32/1 -> out0/1
  enb_counter/1 -> enb_counter_eq_15/1, enb_counter_le_15/1
  nequ_dtc1/1 -> mux/2
  nequ_dtc3/1 -> mux/4
  nequ_dtc6/1 -> mux/7
  nequ_dtc4/1 -> mux/5
  nequ_dtc5/1 -> mux/6
  nequ_dtc9/1 -> mux/10
  nequ_dtc7/1 -> mux/8
  nequ_dtc8/1 -> mux/9
  mux/1 -> Serializer_Subnetwork/1(in0)
  nequ_dtc10/1 -> mux/11
  tapped_delay/1 -> tapped_delay_outunit_delay/1
  nequ_dtc11/1 -> mux/12
  nequ_dtc13/1 -> mux/14
  nequ_dtc15/1 -> mux/16
  nequ_dtc16/1 -> delayMatch/1
  nequ_dtc19/1 -> delayMatch6/1
  nequ_dtc17/1 -> delayMatch1/1
  in3/1 -> nequ_dtc25/1, nequ_dtc24/1, nequ_dtc26/1
  in1/1 -> nequ_dtc18/1, nequ_dtc19/1, nequ_dtc20/1
  in2/1 -> nequ_dtc23/1, nequ_dtc22/1, nequ_dtc21/1
  enb_counter_le_15/1 -> counter/Enable, tapped_delay/2
  delayMatch/1 -> delayMatch3/1
  delayMatch1/1 -> delayMatch4/1
  nequ_dtc18/1 -> delayMatch5/1
  nequ_dtc20/1 -> delayMatch7/1
  nequ_dtc21/1 -> delayMatch8/1
  nequ_dtc24/1 -> delayMatch11/1
  counter_matching_delay/1 -> Serializer_Subnetwork1/2(in1)
  nequ_dtc22/1 -> delayMatch9/1
  nequ_dtc23/1 -> delayMatch10/1
  counter/1(out0) -> counter_matching_delay/1, Serializer_Subnetwork/2(in1)
  nequ_dtc27/1 -> delayMatch14/1
  nequ_dtc25/1 -> delayMatch12/1
  nequ_dtc26/1 -> delayMatch13/1
  nequ_dtc28/1 -> delayMatch15/1
  nequ_dtc29/1 -> delayMatch16/1
  in5/1 -> nequ_dtc31/1, nequ_dtc30/1
  delayMatch13/1 -> mux1/11
  Serializer_Subnetwork/1(out0) -> delayMatch2/1
  delayMatch5/1 -> mux1/3
  delayMatch3/1 -> mux1/1
  delayMatch4/1 -> mux1/2
  delayMatch6/1 -> mux1/4
  delayMatch7/1 -> mux1/5
  delayMatch8/1 -> mux1/6
  delayMatch9/1 -> mux1/7
  delayMatch10/1 -> mux1/8
  delayMatch11/1 -> mux1/9
  delayMatch12/1 -> mux1/10
  delayMatch14/1 -> mux1/12
  delayMatch15/1 -> mux1/13
  delayMatch16/1 -> mux1/14
  nequ_dtc30/1 -> mux1/15
  nequ_dtc31/1 -> mux1/16
  delayMatch2/1 -> delayMatch17/1
  mux1/1 -> Serializer_Subnetwork1/1(in0)
  delayMatch17/1 -> b0_1/1
  Serializer_Subnetwork1/1(out0) -> b0_1/2
  b0_1/1 -> tapped_delay/1
  enb_counter_eq_15/1 -> tapped_delay_outunit_delay/2
  tapped_delay_outunit_delay/1 -> demux/1
  demux/1 -> nequ_dtc32/1
  demux/2 -> nequ_dtc33/1
  demux/3 -> nequ_dtc34/1
  demux/4 -> nequ_dtc35/1
  demux/5 -> nequ_dtc36/1
  demux/6 -> nequ_dtc37/1
  demux/7 -> nequ_dtc38/1
  demux/8 -> nequ_dtc39/1
  demux/9 -> nequ_dtc40/1
  demux/10 -> nequ_dtc41/1
  demux/11 -> nequ_dtc42/1
  demux/12 -> nequ_dtc43/1
  demux/13 -> nequ_dtc44/1
  demux/14 -> nequ_dtc45/1
  demux/15 -> nequ_dtc46/1
  demux/16 -> nequ_dtc47/1
  nequ_dtc33/1 -> out1/1
  nequ_dtc34/1 -> out2/1
  nequ_dtc35/1 -> out3/1
  nequ_dtc36/1 -> out4/1
  nequ_dtc37/1 -> out5/1
  nequ_dtc38/1 -> out6/1
  nequ_dtc39/1 -> out7/1
  nequ_dtc40/1 -> out8/1
  nequ_dtc41/1 -> out9/1
  nequ_dtc42/1 -> out10/1
  nequ_dtc43/1 -> out11/1
  nequ_dtc44/1 -> out12/1
  nequ_dtc45/1 -> out13/1
  nequ_dtc46/1 -> out14/1
  nequ_dtc47/1 -> out15/1
